simulink model "PathFollowing"  (R2021b)
settings: Solver=VariableStepAuto  StartTime=0.0  StopTime=180  RelTol=1e-3
libraries: uavalgslib x3, robotcorelib x1, simulink_extras x1, uavutilslib x1
settings Model: Creator=jihoo  LastModifiedBy=jihoo

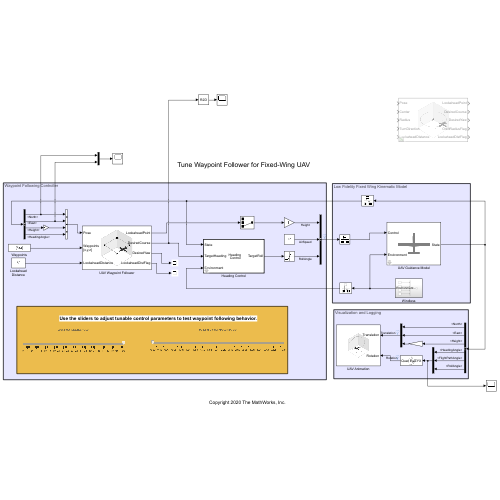
[thumbnail: Simulink's stored preview of the top-level diagram]
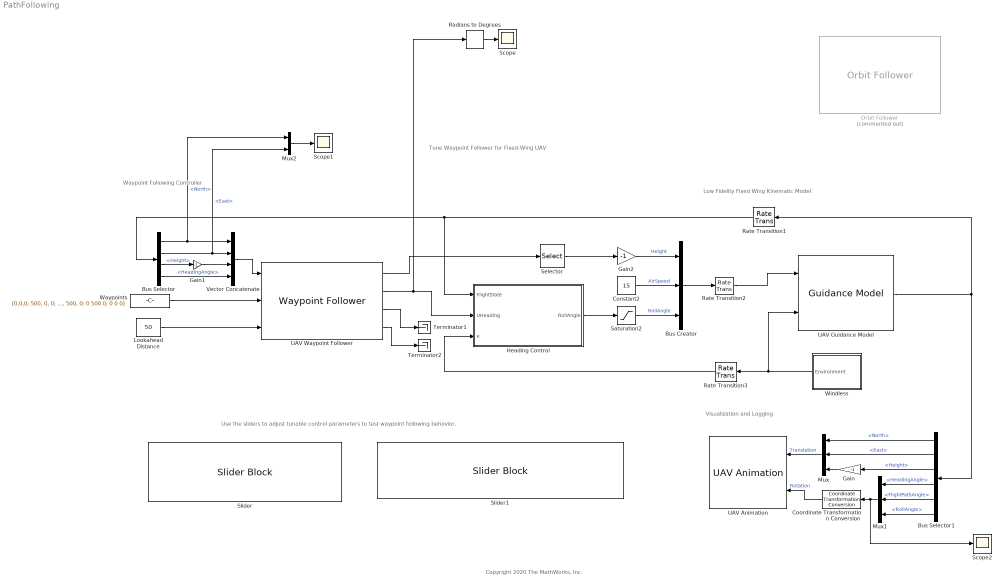
== system PathFollowing ==
  note: Visualization and Logging
  note: Low Fidelity Fixed Wing Kinematic Model
  note: Waypoint Following Controller
  note: Tune Waypoint Follower for Fixed-Wing UAV
  note: Use the sliders to adjust tunable control parameters to test waypoint following behavior.
  note: Copyright 2020 The MathWorks, Inc.
  Bus Creator : BusCreator  Inputs=3  OutDataTypeStr=Bus: FixedWingControlBus  NonVirtualBus=on
  Bus Selector : BusSelector  OutputSignals=North,East,Height,HeadingAngle
  Bus Selector1 : BusSelector  OutputSignals=North,East,Height,HeadingAngle,FlightPathAngle,RollAngle
  Constant2 : Constant  Value=15
  Coordinate Transformation Conversion : robotcorelib/Coordinate Transformation Conversion  InputRepresentation=Euler Angles  InputEulerSequence=ZYX  ShowTrVecInputPort=on  OutputRepresentation=Quaternion  OutputEulerSequence=ZYX  ShowTrVecOutputPort=on  SimulateUsing=Code generation
      settings: SourceProductBaseCode=NV,RO,RR,UV
  Gain : Gain  Gain=-1
  Gain1 : Gain  Gain=-1
  Gain2 : Gain  Gain=-1
  Heading Control : MATLAB Function  TreatAsAtomicUnit=on  mask(Fixed Wing Heading Controller){PHeadingAngle=0.39}
      mask prompts: PHeadingAngle "Heading Control Gain"
      mask help: P controller that regulates fixed wing UAV heading direction through controlling its roll angle. This controller requires that the plane is flying under coordinated flight condition.
  Lookahead Distance : Constant  Value=50
  Mux : Mux  Inputs=3
  Mux1 : Mux  Inputs=3
  Mux2 : Mux  Inputs=2
  Orbit Follower : uavalgslib/Orbit Follower  Commented=on  UAVType=fixed-wing  MinOrbitRadius=1  MinLookaheadDistance=0.1  ExternalReset=none  ShowCrossTrackErrorOutput=off  ShowNumTurnsOutput=off  SimulateUsing=Interpreted execution
      settings: SourceProductBaseCode=UV
  Radians to Degrees : simulink_extras/Transformations/Radians to Degrees
  Rate Transition1 : RateTransition  OutPortSampleTime=0.01
  Rate Transition2 : RateTransition  OutPortSampleTime=0.1
  Rate Transition3 : RateTransition  OutPortSampleTime=0.01
  Saturation2 : Saturate  UpperLimit=20/180*pi  LowerLimit=-20/180*pi
  Scope : Scope
  Scope1 : Scope
  Scope2 : Scope
  Selector : Selector  InputPortWidth=3  IndexOptions=Index vector (dialog)  Indices=[3]  OutputSizes=1
  Slider : SliderBlock  ScaleMin=5  ScaleMax=50
  Slider1 : SliderBlock  ScaleMin=0.39000000000000001  ScaleMax=3.8999999999999999
  Terminator1 : Terminator
  Terminator2 : Terminator
  UAV Animation : uavutilslib/UAV Animation  UAVType=FixedWing  UAVSize=50  InertialZDirection=Down  SampleTime=0.1
      settings: SourceProductBaseCode=UV
  UAV Guidance Model : uavalgslib/Guidance Model  ModelType=FixedWingGuidance  SpecifiedDataType=double  SimulateUsing=Code generation  InitialWorldPositionMultirotor=[0; 0; 0]  InitialWorldVelocityMultirotor=[0; 0; 0]  InitialEulerZYXMultirotor=[0; 0; 0]  InitialBodyAngularRateRPYMultirotor=[0; 0; 0]  InitialThrustMultirotor=0  InitialNorthFixedWing=0  InitialEastFixedWing=0  InitialHeightFixedWing=0  InitialAirSpeedFixedWing=15  InitialHeadingAngleFixedWing=0  InitialFlightPathAngleFixedWing=0  InitialRollAngleFixedWing=0  InitialRollAngleRateFixedWing=0  PDRollMultirotor=[3402.97,116.67]  PDPitchMultirotor=[3402.97, 116.67]  PYawRateMultirotor=1950  PThrustMultirotor=3900  MassMultirotor=0.1  PHeightFixedWing=3.9  PHeadingAngleFixedWing=3.9  PFlightPathAngleFixedWing=39  PDRollFixedWing=[5.9414, 3.9]  PAirSpeedFixedWing=1  FlightPathAngleLimitsFixedWing=[-pi/6, pi/6]  StateBusName='FixedWingStateBus'  ControlBusName='FixedWingControlBus'  EnvironmentBusName='FixedWingEnvironmentBus'  DataType=double
      settings: SourceProductBaseCode=UV
  UAV Waypoint Follower : uavalgslib/Waypoint Follower  UAVType=fixed-wing  StartFrom=first  TransitionRadiusSource=internal  TransitionRadius=10  MinLookaheadDistance=0.1  YawInput=off  ShowCrossTrackErrorOutput=off  ShowStatusOutput=off  SimulateUsing=Code generation
      settings: SourceProductBaseCode=UV
  Vector Concatenate : Concatenate  NumInputs=4
  Waypoints : Constant  Value=[0,0,0; 500, 0, 0; 500, 500, 0; 0 500 0; 0 0 0]  VectorParams1D=off
  Windless : Subsystem  VariantControl=NoWind
  wires:
  Selector/1 -> Gain2/1
  Bus Selector/3 -> Gain1/1  "<Height>"
  Windless/1(Environment) -> UAV Guidance Model/2, Rate Transition3/1
  Bus Selector1/2 -> Mux/2  "<East>"
  UAV Waypoint Follower/4 -> Terminator2/1
  Bus Selector1/3 -> Gain/1  "<Height>"
  UAV Guidance Model/1 -> Bus Selector1/1, Rate Transition1/1
  Mux1/1 -> Scope2/1, Coordinate Transformation Conversion/1
  Bus Creator/1 -> Rate Transition2/1
  Bus Selector1/1 -> Mux/1  "<North>"
  Bus Selector1/4 -> Mux1/1  "<HeadingAngle>"
  Bus Selector/4 -> Vector Concatenate/4  "<HeadingAngle>"
  Rate Transition2/1 -> UAV Guidance Model/1
  Bus Selector1/5 -> Mux1/2  "<FlightPathAngle>"
  Rate Transition3/1 -> Heading Control/3(e)
  Coordinate Transformation Conversion/1 -> UAV Animation/2  "Rotation"
  Mux/1 -> UAV Animation/1  "Translation"
  Vector Concatenate/1 -> UAV Waypoint Follower/1
  Bus Selector/1 -> Mux2/1, Vector Concatenate/1  "<North>"
  Gain1/1 -> Vector Concatenate/3
  Rate Transition1/1 -> Heading Control/1(FlightState), Bus Selector/1
  Bus Selector1/6 -> Mux1/3  "<RollAngle>"
  UAV Waypoint Follower/3 -> Terminator1/1
  UAV Waypoint Follower/2 -> Radians to Degrees/1, Heading Control/2(UHeading)
  UAV Waypoint Follower/1 -> Selector/1
  Saturation2/1 -> Bus Creator/3  "RollAngle"
  Gain/1 -> Mux/3
  Gain2/1 -> Bus Creator/1  "Height"
  Heading Control/1(RollAngle) -> Saturation2/1
  Waypoints/1 -> UAV Waypoint Follower/2
  Lookahead Distance/1 -> UAV Waypoint Follower/3
  Constant2/1 -> Bus Creator/2  "AirSpeed"
  Bus Selector/2 -> Mux2/2, Vector Concatenate/2  "<East>"
  Radians to Degrees/1 -> Scope/1
  Mux2/1 -> Scope1/1

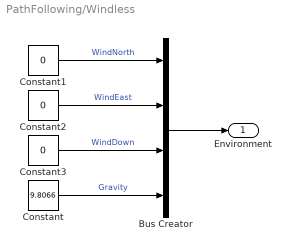
== system PathFollowing/Windless ==
  Bus Creator : BusCreator  Inputs=4  OutDataTypeStr=Bus: FixedWingEnvironmentBus  NonVirtualBus=on
  Constant : Constant  Value=9.8066
  Constant1 : Constant  Value=0
  Constant2 : Constant  Value=0
  Constant3 : Constant  Value=0
  Environment : Outport  VectorParamsAs1DForOutWhenUnconnected=off
  wires:
  Constant2/1 -> Bus Creator/2  "WindEast"
  Constant3/1 -> Bus Creator/3  "WindDown"
  Constant1/1 -> Bus Creator/1  "WindNorth"
  Bus Creator/1 -> Environment/1
  Constant/1 -> Bus Creator/4  "Gravity"

== matlab function PathFollowing/Heading Control ==
  data: FlightState input Bus: FixedWingStateBus; UHeading input; RollAngle output size=[1 1]; e input Bus: FixedWingEnvironmentBus
function RollAngle = fcn(FlightState, UHeading, e)

PHeadingAngle = 0.39;

Va = FlightState.AirSpeed;
HeadingAngle = FlightState.HeadingAngle;
FlightPathAngle = FlightState.FlightPathAngle;

YawAngle = HeadingAngle - asin((1/Va)*[e.WindNorth, e.WindEast]*[-sin(HeadingAngle); cos(HeadingAngle)]);
b = [cos(HeadingAngle)*cos(FlightPathAngle), sin(HeadingAngle)*cos(FlightPathAngle), -sin(FlightPathAngle)]*[e.WindNorth; e.WindEast; e.WindDown];
c = [e.WindNorth, e.WindEast, e.WindDown]*[e.WindNorth; e.WindEast; e.WindDown]- Va^2;
Vg = -b+sqrt(b^2-c);

RollAngle = atan2(PHeadingAngle*angdiff(HeadingAngle,UHeading)*Vg,e.Gravity*cos(HeadingAngle-YawAngle));
